simulink model "DVBS2_LDPC_Decoder_Model"  (R2025b)
settings: Solver=FixedStepDiscrete  StartTime=0  StopTime=simStopTime  FixedStep=1  RelTol=1e-3
libraries: whdledac x1, whdlutilities x1
settings Model: Creator=Ubaid  LastModifiedBy=Ubaid
settings OptimizationCC: BlockReduction=off  ConditionallyExecuteInputs=off

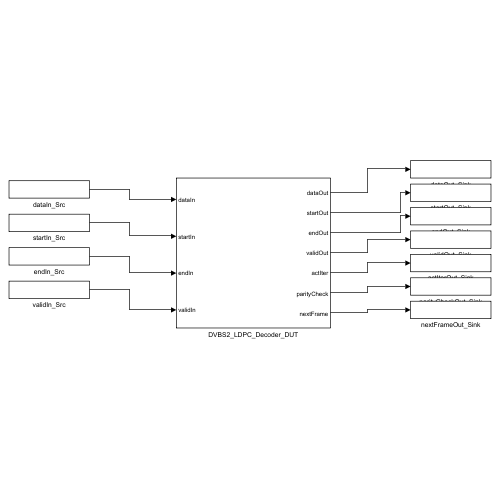
[thumbnail: Simulink's stored preview of the top-level diagram]
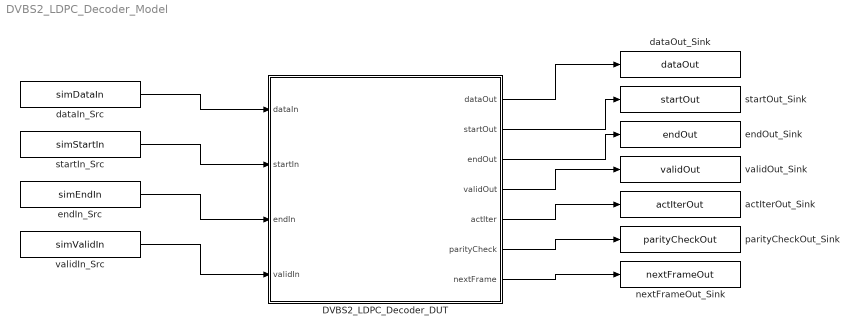
== system DVBS2_LDPC_Decoder_Model ==
  DVBS2_LDPC_Decoder_DUT : Subsystem
  actIterOut_Sink : ToWorkspace  VariableName=actIterOut  SampleTime=-1
  dataIn_Src : FromWorkspace  VariableName=simDataIn  SampleTime=1  Interpolate=off  OutputAfterFinalValue=Setting to zero
  dataOut_Sink : ToWorkspace  VariableName=dataOut  SampleTime=-1
  endIn_Src : FromWorkspace  VariableName=simEndIn  SampleTime=1  Interpolate=off  OutputAfterFinalValue=Setting to zero
  endOut_Sink : ToWorkspace  VariableName=endOut  SampleTime=-1
  nextFrameOut_Sink : ToWorkspace  VariableName=nextFrameOut  SampleTime=-1
  parityCheckOut_Sink : ToWorkspace  VariableName=parityCheckOut  SampleTime=-1
  startIn_Src : FromWorkspace  VariableName=simStartIn  SampleTime=1  Interpolate=off  OutputAfterFinalValue=Setting to zero
  startOut_Sink : ToWorkspace  VariableName=startOut  SampleTime=-1
  validIn_Src : FromWorkspace  VariableName=simValidIn  SampleTime=1  Interpolate=off  OutputAfterFinalValue=Setting to zero
  validOut_Sink : ToWorkspace  VariableName=validOut  SampleTime=-1
  wires:
  dataIn_Src/1 -> DVBS2_LDPC_Decoder_DUT/1(dataIn)
  startIn_Src/1 -> DVBS2_LDPC_Decoder_DUT/2(startIn)
  endIn_Src/1 -> DVBS2_LDPC_Decoder_DUT/3(endIn)
  validIn_Src/1 -> DVBS2_LDPC_Decoder_DUT/4(validIn)
  DVBS2_LDPC_Decoder_DUT/1(dataOut) -> dataOut_Sink/1
  DVBS2_LDPC_Decoder_DUT/2(startOut) -> startOut_Sink/1
  DVBS2_LDPC_Decoder_DUT/3(endOut) -> endOut_Sink/1
  DVBS2_LDPC_Decoder_DUT/4(validOut) -> validOut_Sink/1
  DVBS2_LDPC_Decoder_DUT/5(actIter) -> actIterOut_Sink/1
  DVBS2_LDPC_Decoder_DUT/6(parityCheck) -> parityCheckOut_Sink/1
  DVBS2_LDPC_Decoder_DUT/7(nextFrame) -> nextFrameOut_Sink/1

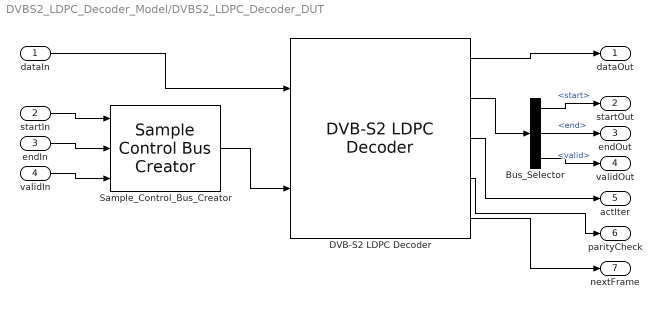
== system DVBS2_LDPC_Decoder_Model/DVBS2_LDPC_Decoder_DUT ==
  dataIn : Inport
  startIn : Inport  Port=2
  endIn : Inport  Port=3
  validIn : Inport  Port=4
  Bus_Selector : BusSelector  OutputSignals=start,end,valid
  DVB-S2 LDPC Decoder : whdledac/DVB-S2 LDPC Decoder  FECFrameSource=Property  FECFrame=Short  CodeRateSource=Property  CodeRateNormal=1/4  CodeRateShort=1/2  Parallelism=45  Algorithm=Normalized min-sum  SourceScalingFactor=Property  ScalingFactor=0.75  Termination=Early  SpecifyInputs=Property  NumIterations=8  MaxNumIterations=8  ParityCheckStatus=on  SimulateUsing=Code generation
  Sample_Control_Bus_Creator : whdlutilities/Sample Control Bus Creator
  dataOut : Outport
  startOut : Outport  Port=2
  endOut : Outport  Port=3
  validOut : Outport  Port=4
  actIter : Outport  Port=5
  parityCheck : Outport  Port=6
  nextFrame : Outport  Port=7
  wires:
  startIn/1 -> Sample_Control_Bus_Creator/1
  endIn/1 -> Sample_Control_Bus_Creator/2
  validIn/1 -> Sample_Control_Bus_Creator/3
  dataIn/1 -> DVB-S2 LDPC Decoder/1
  Sample_Control_Bus_Creator/1 -> DVB-S2 LDPC Decoder/2
  DVB-S2 LDPC Decoder/1 -> dataOut/1
  DVB-S2 LDPC Decoder/2 -> Bus_Selector/1
  DVB-S2 LDPC Decoder/3 -> actIter/1
  DVB-S2 LDPC Decoder/4 -> parityCheck/1
  DVB-S2 LDPC Decoder/5 -> nextFrame/1
  Bus_Selector/1 -> startOut/1  "<start>"
  Bus_Selector/2 -> endOut/1  "<end>"
  Bus_Selector/3 -> validOut/1  "<valid>"
